simulink model "fft_biplex_test"  (Simulink 7.4)
settings: Solver=VariableStepDiscrete  StartTime=0.0  StopTime=2000  RelTol=1e-3
libraries: xbsIndex_r4 x808, casper_library_misc x46, casper_library_delays x10, casper_library_reorder x2, casper_library_ffts_twiddle x1
(part 2 of 8)

== system fft_biplex_test/fft_biplex/biplex_core/fft_stage_1 ==
  in1 : Inport  OutDataType=sfix(16)  OutScaling=2^0
  in2 : Inport  Port=2  OutDataType=sfix(16)  OutScaling=2^0
  of_in : Inport  Port=3  OutDataType=sfix(16)  OutScaling=2^0
  sync : Inport  Port=4  OutDataType=sfix(16)  OutScaling=2^0
  shift : Inport  Port=5  OutDataType=sfix(16)  OutScaling=2^0
  Counter : xbsIndex_r4/Counter  cnt_type=Free Running  cnt_to=Inf  operation=Up  start_count=0  cnt_by_val=1  arith_type=Unsigned  n_bits=FFTSize-FFTStage+1  bin_pt=0  load_pin=off  rst=on  en=off  explicit_period=off  period=1  dbl_ovrd=off  use_behavioral_HDL=off  implementation=Fabric  use_rpm=off  block_type=counter
      settings: xl_area=[0, 0, 0, 0, 0, 0, 0]  block_version=9.1.01
  Delay : xbsIndex_r4/Delay  en=off  latency=1  dbl_ovrd=off  reg_retiming=off  block_type=delay
      settings: xl_area=[0, 0, 0, 0, 0, 0, 0]  block_version=9.1.01
  Logical1 : xbsIndex_r4/Logical  logical_function=OR  inputs=2  en=off  latency=1  precision=Full  arith_type=Unsigned  n_bits=8  bin_pt=2  align_bp=on  dbl_ovrd=off  block_type=logical
      settings: xl_area=[0, 0, 0, 0, 0, 0, 0]  block_version=9.1.01
  Mux : xbsIndex_r4/Mux  inputs=2  en=off  latency=1  precision=Full  arith_type="Signed  (2's comp)"  n_bits=8  bin_pt=2  quantization=Truncate  overflow=Wrap  dbl_ovrd=off  block_type=mux
      settings: xl_area=[0, 0, 0, 0, 0, 0, 0]  block_version=9.1.01
  Mux1 : xbsIndex_r4/Mux  inputs=2  en=off  latency=1  precision=Full  arith_type="Signed  (2's comp)"  n_bits=8  bin_pt=2  quantization=Truncate  overflow=Wrap  dbl_ovrd=off  block_type=mux
      settings: xl_area=[0, 0, 0, 0, 0, 0, 0]  block_version=9.1.01
  Slice : xbsIndex_r4/Slice  nbits=1  boolean_output=on  mode=Lower Bit Location + Width  bit1=-(FFTStage - 1)  base1=MSB of Input  bit0=FFTStage - 1  base0=LSB of Input  dbl_ovrd=off  block_type=slice
      settings: infoedit="Extracts a given range of bits from each input sample and presents it at the output.  The output type is ordinarily unsigned with binary point at zero, but can be Boolean when the slice is one bit wide.<P><P>Hardware notes: In hardware this block costs nothing."  block_version=9.1.01
  Slice1 : xbsIndex_r4/Slice  nbits=1  boolean_output=off  mode=Upper Bit Location + Width  bit1=0  base1=MSB of Input  bit0=0  base0=LSB of Input  dbl_ovrd=off  block_type=slice
      settings: infoedit="Extracts a given range of bits from each input sample and presents it at the output.  The output type is ordinarily unsigned with binary point at zero, but can be Boolean when the slice is one bit wide.<P><P>Hardware notes: In hardware this block costs nothing."  block_version=9.1.01
  butterfly_direct : Subsystem  AncestorBlock=casper_library_ffts/butterfly_direct  mask(butterfly_direct){biplex=on, FFTSize=8, Coeffs=0, StepPeriod=7, coeff_bit_width=12, input_bit_width=12, downshift=off, add_latency=2, mult_latency=3, bram_latency=2, conv_latency=2, quantization=Round  (unbiased: +/- Inf), overflow=Saturate, arch=Virtex2Pro, opt_target=multipliers, coeffs_bram=off, use_hdl=on, use_embedded=off, hardcode_shifts=off, dsp48_adders=off}
      mask prompts: biplex "Used in biplex FFT"; FFTSize "Size of FFT: (2^? pts)"; Coeffs "Coefficients: (0 to 2^(FFTSize-1)-1)"; StepPeriod "Coefficient Step Period: (2^?)"; coeff_bit_width "Coefficient Bit Width"; input_bit_width "Input/Output Bit Width:"; add_latency "Add Latency"; mult_latency "Mult Latency"; bram_latency "BRAM Latency"; conv_latency "Convert latency"; quantization "Quantization Behavior"; overflow "Overflow Behavior"; arch "Architecture"; opt_target "Use less"; coeffs_bram "Store coefficients in BRAM"; use_hdl "Use behavioural HDL for multipliers"; use_embedded "Use embedded multipliers"; hardcode_shifts "Hardcode shift schedule"; dsp48_adders "Use DSP48s for adders"
      mask help: FFT internal block.
      mask init:
      | butterfly_direct_init(gcb, ...
      |     'biplex', biplex, ...
      |     'FFTSize', FFTSize, ...
      |     'Coeffs', Coeffs, ...
      |     'StepPeriod', StepPeriod, ...
      |     'coeff_bit_width', coeff_bit_width, ...
      |     'input_bit_width', input_bit_width, ...
      |     'hardcode_shifts', hardcode_shifts, ...
      |     'downshift', downshift, ...
      |     'add_latency', add_latency, ...
      |     'mult_latency', mult_latency, ...
      |     'bram_latency', bram_latency, ...
      |     'conv_latency', conv_latency, ...
      |     'quantization', quantization, ...
      |     'overflow', overflow, ...
      |     'arch', arch, ...
      |     'opt_target', opt_target, ...
      |     'coeffs_bram', coeffs_bram, ...    
      |     'use_hdl', use_hdl, ...
      |     'use_embedded', use_embedded, ...
      |     'dsp48_adders', dsp48_adders);
      settings: AttributesFormatString=|
      | twiddle_pass_through
      | coeffs in slices
      mask StyleString: checkbox,edit,edit,edit,edit,edit,checkbox,edit,edit,edit,edit,popup(Truncate|Round  (unbiased: +/- Inf)|Round  (unbiased: Even Values)),popup(Wrap|Saturate|Error),popup(Virtex2Pro|Virtex5),popup(logic|multipliers),checkbox,checkbox,checkbox,checkbox,checkbox
      mask CallbackString:
      | ||Coeffs = get_param(gcb, 'Coeffs');
      | if (length(eval(Coeffs)) == 1),
      |     set_param_state(gcb, 'StepPeriod', 'off');
      |     set_param_state(gcb, 'coeffs_bram', 'off');
      |     set_param_state(gcb, 'coeff_bit_width', 'off');
      | else
      |     set_param_state(gcb, 'StepPeriod', 'on');
      |     set_param_state(gcb, 'coeffs_bram', 'on');
      |     set_param_state(gcb, 'coeff_bit_width', 'on');
      | end|||||||||||fft_callback_arch(gcb);|||% make mutually exclusive with use_embedded.
      | 
      | use_hdl = get_param(gcb, 'use_hdl');
      | if strcmp(use_hdl, 'on'),
      |     set_param_state(gcb, 'use_embedded', 'off');
      | else
      |     set_param_state(gcb, 'use_embedded', 'on');
      | end|% make mutually exclusive with use_hdl.
      | 
      | use_hdl = get_param(gcb, 'use_embedded');
      | if strcmp(use_hdl, 'on'),
      |     set_param_state(gcb, 'use_hdl', 'off');
      | else
      |     set_param_state(gcb, 'use_hdl', 'on');
      | end|hardcode_shifts = get_param(gcb, 'hardcode_shifts');
      | set_param_state(gcb, 'downshift', hardcode_shifts);|fft_callback_dsp48_adders(gcb);
      mask TabNameString: Basic,Basic,Basic,Basic,Basic,Basic,Basic,Latency,Latency,Latency,Latency,Implementation,Implementation,Implementation,Implementation,Implementation,Implementation,Implementation,Implementation,Implementation
  delay_b : Subsystem  AncestorBlock=casper_library_delays/delay_bram  mask(delay_bram){DelayLen=2^(FFTSize-FFTStage), bram_latency=bram_latency, use_dsp48=off}
      mask prompts: DelayLen "Delay By:"; bram_latency "BRAM Latency"; use_dsp48 "Use DSP48"
      mask help: A delay block that uses BRAM for its storage.
      mask init:
      | if (DelayLen <= bram_latency)
      | 	error('delay value must be greater than BRAM Latency');
      | end
      | BitWidth = max(ceil(log2(DelayLen)), 2);
      | if strcmp(use_dsp48,'on'),
      |     set_param([gcb,'/Counter'], 'use_behavioral_HDL', 'off', ...
      |         'use_rpm', 'on', 'implementation', 'DSP48');
      | else, %default counter settings
      |         set_param([gcb,'/Counter'], 'use_behavioral_HDL', 'off', ...
      |         'use_rpm', 'off', 'implementation', 'Fabric');
      | end
      mask Help: eval('xlWeb(''http://casper.berkeley.edu/wiki/Delay_bram'')')
  delay_f : Subsystem  AncestorBlock=casper_library_delays/delay_bram  mask(delay_bram){DelayLen=2^(FFTSize-FFTStage), bram_latency=bram_latency, use_dsp48=off}
      mask prompts: DelayLen "Delay By:"; bram_latency "BRAM Latency"; use_dsp48 "Use DSP48"
      mask help: A delay block that uses BRAM for its storage.
      mask init: same as fft_biplex_test/fft_biplex/biplex_core/fft_stage_1/delay_b
      mask Help: eval('xlWeb(''http://casper.berkeley.edu/wiki/Delay_bram'')')
  sync_delay : casper_library_delays/sync_delay  SystemSampleTime=-1  DelayLen=2^(FFTSize - FFTStage)
  out1 : Outport  OutDataType=sfix(16)  OutScaling=2^0
  out2 : Outport  Port=2  OutDataType=sfix(16)  OutScaling=2^0
  of : Outport  Port=3  OutDataType=sfix(16)  OutScaling=2^0
  sync_out : Outport  Port=4  OutDataType=sfix(16)  OutScaling=2^0
  wires:
  butterfly_direct/4(sync_out) -> sync_out/1
  butterfly_direct/3(of) -> Logical1/1
  butterfly_direct/2(a-bw) -> out2/1
  butterfly_direct/1(a+bw) -> out1/1
  Slice/1 -> butterfly_direct/4(shift)
  sync_delay/1 -> butterfly_direct/3(sync)
  delay_b/1(Out1) -> butterfly_direct/1(a)
  in2/1 -> delay_f/1(In1)
  Slice1/1 -> Mux1/1, Mux/1
  in1/1 -> Mux1/2, Mux/3
  delay_f/1(Out1) -> Mux/2, Mux1/3
  Mux1/1 -> delay_b/1(In1)
  Mux/1 -> butterfly_direct/2(b)
  Counter/1 -> Slice1/1
  sync/1 -> Delay/1, Counter/1
  Delay/1 -> sync_delay/1
  Logical1/1 -> of/1
  of_in/1 -> Logical1/2
  shift/1 -> Slice/1

== system fft_biplex_test/fft_biplex/biplex_core/fft_stage_2 ==
  in1 : Inport  OutDataType=sfix(16)  OutScaling=2^0
  in2 : Inport  Port=2  OutDataType=sfix(16)  OutScaling=2^0
  of_in : Inport  Port=3  OutDataType=sfix(16)  OutScaling=2^0
  sync : Inport  Port=4  OutDataType=sfix(16)  OutScaling=2^0
  shift : Inport  Port=5  OutDataType=sfix(16)  OutScaling=2^0
  Counter : xbsIndex_r4/Counter  cnt_type=Free Running  cnt_to=Inf  operation=Up  start_count=0  cnt_by_val=1  arith_type=Unsigned  n_bits=FFTSize-FFTStage+1  bin_pt=0  load_pin=off  rst=on  en=off  explicit_period=off  period=1  dbl_ovrd=off  use_behavioral_HDL=off  implementation=Fabric  use_rpm=off  block_type=counter
      settings: xl_area=[0, 0, 0, 0, 0, 0, 0]  block_version=9.1.01
  Delay : xbsIndex_r4/Delay  en=off  latency=1  dbl_ovrd=off  reg_retiming=off  block_type=delay
      settings: xl_area=[0, 0, 0, 0, 0, 0, 0]  block_version=9.1.01
  Logical1 : xbsIndex_r4/Logical  logical_function=OR  inputs=2  en=off  latency=1  precision=Full  arith_type=Unsigned  n_bits=8  bin_pt=2  align_bp=on  dbl_ovrd=off  block_type=logical
      settings: xl_area=[0, 0, 0, 0, 0, 0, 0]  block_version=9.1.01
  Mux : xbsIndex_r4/Mux  inputs=2  en=off  latency=1  precision=Full  arith_type="Signed  (2's comp)"  n_bits=8  bin_pt=2  quantization=Truncate  overflow=Wrap  dbl_ovrd=off  block_type=mux
      settings: xl_area=[0, 0, 0, 0, 0, 0, 0]  block_version=9.1.01
  Mux1 : xbsIndex_r4/Mux  inputs=2  en=off  latency=1  precision=Full  arith_type="Signed  (2's comp)"  n_bits=8  bin_pt=2  quantization=Truncate  overflow=Wrap  dbl_ovrd=off  block_type=mux
      settings: xl_area=[0, 0, 0, 0, 0, 0, 0]  block_version=9.1.01
  Slice : xbsIndex_r4/Slice  nbits=1  boolean_output=on  mode=Lower Bit Location + Width  bit1=-(FFTStage - 1)  base1=MSB of Input  bit0=FFTStage - 1  base0=LSB of Input  dbl_ovrd=off  block_type=slice
      settings: infoedit="Extracts a given range of bits from each input sample and presents it at the output.  The output type is ordinarily unsigned with binary point at zero, but can be Boolean when the slice is one bit wide.<P><P>Hardware notes: In hardware this block costs nothing."  block_version=9.1.01
  Slice1 : xbsIndex_r4/Slice  nbits=1  boolean_output=off  mode=Upper Bit Location + Width  bit1=0  base1=MSB of Input  bit0=0  base0=LSB of Input  dbl_ovrd=off  block_type=slice
      settings: infoedit="Extracts a given range of bits from each input sample and presents it at the output.  The output type is ordinarily unsigned with binary point at zero, but can be Boolean when the slice is one bit wide.<P><P>Hardware notes: In hardware this block costs nothing."  block_version=9.1.01
  butterfly_direct : Subsystem  AncestorBlock=casper_library_ffts/butterfly_direct  mask(butterfly_direct){biplex=on, FFTSize=8, Coeffs=[0                                      1], StepPeriod=6, coeff_bit_width=12, input_bit_width=12, downshift=off, add_latency=2, mult_latency=3, bram_latency=2, conv_latency=2, quantization=Round  (unbiased: +/- Inf), overflow=Saturate, arch=Virtex2Pro, opt_target=multipliers, coeffs_bram=off, use_hdl=on, use_embedded=off, hardcode_shifts=off, dsp48_adders=off}
      mask prompts: biplex "Used in biplex FFT"; FFTSize "Size of FFT: (2^? pts)"; Coeffs "Coefficients: (0 to 2^(FFTSize-1)-1)"; StepPeriod "Coefficient Step Period: (2^?)"; coeff_bit_width "Coefficient Bit Width"; input_bit_width "Input/Output Bit Width:"; add_latency "Add Latency"; mult_latency "Mult Latency"; bram_latency "BRAM Latency"; conv_latency "Convert latency"; quantization "Quantization Behavior"; overflow "Overflow Behavior"; arch "Architecture"; opt_target "Use less"; coeffs_bram "Store coefficients in BRAM"; use_hdl "Use behavioural HDL for multipliers"; use_embedded "Use embedded multipliers"; hardcode_shifts "Hardcode shift schedule"; dsp48_adders "Use DSP48s for adders"
      mask help: FFT internal block.
      mask init: same as fft_biplex_test/fft_biplex/biplex_core/fft_stage_1/butterfly_direct
      settings: AttributesFormatString=|
      | twiddle_stage_2
      | coeffs in slices
      mask StyleString: checkbox,edit,edit,edit,edit,edit,checkbox,edit,edit,edit,edit,popup(Truncate|Round  (unbiased: +/- Inf)|Round  (unbiased: Even Values)),popup(Wrap|Saturate|Error),popup(Virtex2Pro|Virtex5),popup(logic|multipliers),checkbox,checkbox,checkbox,checkbox,checkbox
      mask CallbackString:
      | ||Coeffs = get_param(gcb, 'Coeffs');
      | if (length(eval(Coeffs)) == 1),
      |     set_param_state(gcb, 'StepPeriod', 'off');
      |     set_param_state(gcb, 'coeffs_bram', 'off');
      |     set_param_state(gcb, 'coeff_bit_width', 'off');
      | else
      |     set_param_state(gcb, 'StepPeriod', 'on');
      |     set_param_state(gcb, 'coeffs_bram', 'on');
      |     set_param_state(gcb, 'coeff_bit_width', 'on');
      | end|||||||||||fft_callback_arch(gcb);|||% make mutually exclusive with use_embedded.
      | 
      | use_hdl = get_param(gcb, 'use_hdl');
      | if strcmp(use_hdl, 'on'),
      |     set_param_state(gcb, 'use_embedded', 'off');
      | else
      |     set_param_state(gcb, 'use_embedded', 'on');
      | end|% make mutually exclusive with use_hdl.
      | 
      | use_hdl = get_param(gcb, 'use_embedded');
      | if strcmp(use_hdl, 'on'),
      |     set_param_state(gcb, 'use_hdl', 'off');
      | else
      |     set_param_state(gcb, 'use_hdl', 'on');
      | end|hardcode_shifts = get_param(gcb, 'hardcode_shifts');
      | set_param_state(gcb, 'downshift', hardcode_shifts);|fft_callback_dsp48_adders(gcb);
      mask TabNameString: Basic,Basic,Basic,Basic,Basic,Basic,Basic,Latency,Latency,Latency,Latency,Implementation,Implementation,Implementation,Implementation,Implementation,Implementation,Implementation,Implementation,Implementation
  delay_b : Subsystem  AncestorBlock=casper_library_delays/delay_bram  mask(delay_bram){DelayLen=2^(FFTSize-FFTStage), bram_latency=bram_latency, use_dsp48=off}
      mask prompts: DelayLen "Delay By:"; bram_latency "BRAM Latency"; use_dsp48 "Use DSP48"
      mask help: A delay block that uses BRAM for its storage.
      mask init: same as fft_biplex_test/fft_biplex/biplex_core/fft_stage_1/delay_b
      mask Help: eval('xlWeb(''http://casper.berkeley.edu/wiki/Delay_bram'')')
  delay_f : Subsystem  AncestorBlock=casper_library_delays/delay_bram  mask(delay_bram){DelayLen=2^(FFTSize-FFTStage), bram_latency=bram_latency, use_dsp48=off}
      mask prompts: DelayLen "Delay By:"; bram_latency "BRAM Latency"; use_dsp48 "Use DSP48"
      mask help: A delay block that uses BRAM for its storage.
      mask init: same as fft_biplex_test/fft_biplex/biplex_core/fft_stage_1/delay_b
      mask Help: eval('xlWeb(''http://casper.berkeley.edu/wiki/Delay_bram'')')
  sync_delay : casper_library_delays/sync_delay  SystemSampleTime=-1  DelayLen=2^(FFTSize - FFTStage)
  out1 : Outport  OutDataType=sfix(16)  OutScaling=2^0
  out2 : Outport  Port=2  OutDataType=sfix(16)  OutScaling=2^0
  of : Outport  Port=3  OutDataType=sfix(16)  OutScaling=2^0
  sync_out : Outport  Port=4  OutDataType=sfix(16)  OutScaling=2^0
  wires:
  butterfly_direct/4(sync_out) -> sync_out/1
  butterfly_direct/3(of) -> Logical1/1
  butterfly_direct/2(a-bw) -> out2/1
  butterfly_direct/1(a+bw) -> out1/1
  Slice/1 -> butterfly_direct/4(shift)
  sync_delay/1 -> butterfly_direct/3(sync)
  delay_b/1(Out1) -> butterfly_direct/1(a)
  in2/1 -> delay_f/1(In1)
  Slice1/1 -> Mux1/1, Mux/1
  in1/1 -> Mux1/2, Mux/3
  delay_f/1(Out1) -> Mux/2, Mux1/3
  Mux1/1 -> delay_b/1(In1)
  Mux/1 -> butterfly_direct/2(b)
  Counter/1 -> Slice1/1
  sync/1 -> Delay/1, Counter/1
  Delay/1 -> sync_delay/1
  Logical1/1 -> of/1
  of_in/1 -> Logical1/2
  shift/1 -> Slice/1

== system fft_biplex_test/fft_biplex/biplex_core/fft_stage_3 ==
  in1 : Inport  OutDataType=sfix(16)  OutScaling=2^0
  in2 : Inport  Port=2  OutDataType=sfix(16)  OutScaling=2^0
  of_in : Inport  Port=3  OutDataType=sfix(16)  OutScaling=2^0
  sync : Inport  Port=4  OutDataType=sfix(16)  OutScaling=2^0
  shift : Inport  Port=5  OutDataType=sfix(16)  OutScaling=2^0
  Counter : xbsIndex_r4/Counter  cnt_type=Free Running  cnt_to=Inf  operation=Up  start_count=0  cnt_by_val=1  arith_type=Unsigned  n_bits=FFTSize-FFTStage+1  bin_pt=0  load_pin=off  rst=on  en=off  explicit_period=off  period=1  dbl_ovrd=off  use_behavioral_HDL=off  implementation=Fabric  use_rpm=off  block_type=counter
      settings: xl_area=[0, 0, 0, 0, 0, 0, 0]  block_version=9.1.01
  Delay : xbsIndex_r4/Delay  en=off  latency=1  dbl_ovrd=off  reg_retiming=off  block_type=delay
      settings: xl_area=[0, 0, 0, 0, 0, 0, 0]  block_version=9.1.01
  Logical1 : xbsIndex_r4/Logical  logical_function=OR  inputs=2  en=off  latency=1  precision=Full  arith_type=Unsigned  n_bits=8  bin_pt=2  align_bp=on  dbl_ovrd=off  block_type=logical
      settings: xl_area=[0, 0, 0, 0, 0, 0, 0]  block_version=9.1.01
  Mux : xbsIndex_r4/Mux  inputs=2  en=off  latency=1  precision=Full  arith_type="Signed  (2's comp)"  n_bits=8  bin_pt=2  quantization=Truncate  overflow=Wrap  dbl_ovrd=off  block_type=mux
      settings: xl_area=[0, 0, 0, 0, 0, 0, 0]  block_version=9.1.01
  Mux1 : xbsIndex_r4/Mux  inputs=2  en=off  latency=1  precision=Full  arith_type="Signed  (2's comp)"  n_bits=8  bin_pt=2  quantization=Truncate  overflow=Wrap  dbl_ovrd=off  block_type=mux
      settings: xl_area=[0, 0, 0, 0, 0, 0, 0]  block_version=9.1.01
  Slice : xbsIndex_r4/Slice  nbits=1  boolean_output=on  mode=Lower Bit Location + Width  bit1=-(FFTStage - 1)  base1=MSB of Input  bit0=FFTStage - 1  base0=LSB of Input  dbl_ovrd=off  block_type=slice
      settings: infoedit="Extracts a given range of bits from each input sample and presents it at the output.  The output type is ordinarily unsigned with binary point at zero, but can be Boolean when the slice is one bit wide.<P><P>Hardware notes: In hardware this block costs nothing."  block_version=9.1.01
  Slice1 : xbsIndex_r4/Slice  nbits=1  boolean_output=off  mode=Upper Bit Location + Width  bit1=0  base1=MSB of Input  bit0=0  base0=LSB of Input  dbl_ovrd=off  block_type=slice
      settings: infoedit="Extracts a given range of bits from each input sample and presents it at the output.  The output type is ordinarily unsigned with binary point at zero, but can be Boolean when the slice is one bit wide.<P><P>Hardware notes: In hardware this block costs nothing."  block_version=9.1.01
  butterfly_direct : Subsystem  AncestorBlock=casper_library_ffts/butterfly_direct  mask(butterfly_direct){biplex=on, FFTSize=8, Coeffs=getfield( getfield( get_param( gcb,'UserData' ), 'parameters'),'Coeffs'), StepPeriod=5, coeff_bit_width=12, input_bit_width=12, downshift=off, add_latency=2, mult_latency=3, bram_latency=2, conv_latency=2, quantization=Round  (unbiased: +/- Inf), overflow=Saturate, arch=Virtex2Pro, opt_target=multipliers, coeffs_bram=on, use_hdl=on, use_embedded=off, hardcode_shifts=off, dsp48_adders=off}
      mask prompts: biplex "Used in biplex FFT"; FFTSize "Size of FFT: (2^? pts)"; Coeffs "Coefficients: (0 to 2^(FFTSize-1)-1)"; StepPeriod "Coefficient Step Period: (2^?)"; coeff_bit_width "Coefficient Bit Width"; input_bit_width "Input/Output Bit Width:"; add_latency "Add Latency"; mult_latency "Mult Latency"; bram_latency "BRAM Latency"; conv_latency "Convert latency"; quantization "Quantization Behavior"; overflow "Overflow Behavior"; arch "Architecture"; opt_target "Use less"; coeffs_bram "Store coefficients in BRAM"; use_hdl "Use behavioural HDL for multipliers"; use_embedded "Use embedded multipliers"; hardcode_shifts "Hardcode shift schedule"; dsp48_adders "Use DSP48s for adders"
      mask help: FFT internal block.
      mask init: same as fft_biplex_test/fft_biplex/biplex_core/fft_stage_1/butterfly_direct
      settings: AttributesFormatString=|
      | twiddle_general_3mult
      | coeffs in BRAM
      mask StyleString: checkbox,edit,edit,edit,edit,edit,checkbox,edit,edit,edit,edit,popup(Truncate|Round  (unbiased: +/- Inf)|Round  (unbiased: Even Values)),popup(Wrap|Saturate|Error),popup(Virtex2Pro|Virtex5),popup(logic|multipliers),checkbox,checkbox,checkbox,checkbox,checkbox
      mask CallbackString:
      | ||Coeffs = get_param(gcb, 'Coeffs');
      | if (length(eval(Coeffs)) == 1),
      |     set_param_state(gcb, 'StepPeriod', 'off');
      |     set_param_state(gcb, 'coeffs_bram', 'off');
      |     set_param_state(gcb, 'coeff_bit_width', 'off');
      | else
      |     set_param_state(gcb, 'StepPeriod', 'on');
      |     set_param_state(gcb, 'coeffs_bram', 'on');
      |     set_param_state(gcb, 'coeff_bit_width', 'on');
      | end|||||||||||fft_callback_arch(gcb);|||% make mutually exclusive with use_embedded.
      | 
      | use_hdl = get_param(gcb, 'use_hdl');
      | if strcmp(use_hdl, 'on'),
      |     set_param_state(gcb, 'use_embedded', 'off');
      | else
      |     set_param_state(gcb, 'use_embedded', 'on');
      | end|% make mutually exclusive with use_hdl.
      | 
      | use_hdl = get_param(gcb, 'use_embedded');
      | if strcmp(use_hdl, 'on'),
      |     set_param_state(gcb, 'use_hdl', 'off');
      | else
      |     set_param_state(gcb, 'use_hdl', 'on');
      | end|hardcode_shifts = get_param(gcb, 'hardcode_shifts');
      | set_param_state(gcb, 'downshift', hardcode_shifts);|fft_callback_dsp48_adders(gcb);
      mask TabNameString: Basic,Basic,Basic,Basic,Basic,Basic,Basic,Latency,Latency,Latency,Latency,Implementation,Implementation,Implementation,Implementation,Implementation,Implementation,Implementation,Implementation,Implementation
  delay_b : Subsystem  AncestorBlock=casper_library_delays/delay_bram  mask(delay_bram){DelayLen=2^(FFTSize-FFTStage), bram_latency=bram_latency, use_dsp48=off}
      mask prompts: DelayLen "Delay By:"; bram_latency "BRAM Latency"; use_dsp48 "Use DSP48"
      mask help: A delay block that uses BRAM for its storage.
      mask init: same as fft_biplex_test/fft_biplex/biplex_core/fft_stage_1/delay_b
      mask Help: eval('xlWeb(''http://casper.berkeley.edu/wiki/Delay_bram'')')
  delay_f : Subsystem  AncestorBlock=casper_library_delays/delay_bram  mask(delay_bram){DelayLen=2^(FFTSize-FFTStage), bram_latency=bram_latency, use_dsp48=off}
      mask prompts: DelayLen "Delay By:"; bram_latency "BRAM Latency"; use_dsp48 "Use DSP48"
      mask help: A delay block that uses BRAM for its storage.
      mask init: same as fft_biplex_test/fft_biplex/biplex_core/fft_stage_1/delay_b
      mask Help: eval('xlWeb(''http://casper.berkeley.edu/wiki/Delay_bram'')')
  sync_delay : casper_library_delays/sync_delay  SystemSampleTime=-1  DelayLen=2^(FFTSize - FFTStage)
  out1 : Outport  OutDataType=sfix(16)  OutScaling=2^0
  out2 : Outport  Port=2  OutDataType=sfix(16)  OutScaling=2^0
  of : Outport  Port=3  OutDataType=sfix(16)  OutScaling=2^0
  sync_out : Outport  Port=4  OutDataType=sfix(16)  OutScaling=2^0
  wires:
  shift/1 -> Slice/1
  of_in/1 -> Logical1/2
  Logical1/1 -> of/1
  Delay/1 -> sync_delay/1
  sync/1 -> Counter/1, Delay/1
  Counter/1 -> Slice1/1
  Mux/1 -> butterfly_direct/2(b)
  Mux1/1 -> delay_b/1(In1)
  delay_f/1(Out1) -> Mux1/3, Mux/2
  in1/1 -> Mux/3, Mux1/2
  Slice1/1 -> Mux/1, Mux1/1
  in2/1 -> delay_f/1(In1)
  delay_b/1(Out1) -> butterfly_direct/1(a)
  sync_delay/1 -> butterfly_direct/3(sync)
  Slice/1 -> butterfly_direct/4(shift)
  butterfly_direct/1(a+bw) -> out1/1
  butterfly_direct/2(a-bw) -> out2/1
  butterfly_direct/3(of) -> Logical1/1
  butterfly_direct/4(sync_out) -> sync_out/1

== system fft_biplex_test/fft_biplex/biplex_core/fft_stage_4 ==
  in1 : Inport  OutDataType=sfix(16)  OutScaling=2^0
  in2 : Inport  Port=2  OutDataType=sfix(16)  OutScaling=2^0
  of_in : Inport  Port=3  OutDataType=sfix(16)  OutScaling=2^0
  sync : Inport  Port=4  OutDataType=sfix(16)  OutScaling=2^0
  shift : Inport  Port=5  OutDataType=sfix(16)  OutScaling=2^0
  Counter : xbsIndex_r4/Counter  cnt_type=Free Running  cnt_to=Inf  operation=Up  start_count=0  cnt_by_val=1  arith_type=Unsigned  n_bits=FFTSize-FFTStage+1  bin_pt=0  load_pin=off  rst=on  en=off  explicit_period=off  period=1  dbl_ovrd=off  use_behavioral_HDL=off  implementation=Fabric  use_rpm=off  block_type=counter
      settings: xl_area=[0, 0, 0, 0, 0, 0, 0]  block_version=9.1.01
  Delay : xbsIndex_r4/Delay  en=off  latency=1  dbl_ovrd=off  reg_retiming=off  block_type=delay
      settings: xl_area=[0, 0, 0, 0, 0, 0, 0]  block_version=9.1.01
  Logical1 : xbsIndex_r4/Logical  logical_function=OR  inputs=2  en=off  latency=1  precision=Full  arith_type=Unsigned  n_bits=8  bin_pt=2  align_bp=on  dbl_ovrd=off  block_type=logical
      settings: xl_area=[0, 0, 0, 0, 0, 0, 0]  block_version=9.1.01
  Mux : xbsIndex_r4/Mux  inputs=2  en=off  latency=1  precision=Full  arith_type="Signed  (2's comp)"  n_bits=8  bin_pt=2  quantization=Truncate  overflow=Wrap  dbl_ovrd=off  block_type=mux
      settings: xl_area=[0, 0, 0, 0, 0, 0, 0]  block_version=9.1.01
  Mux1 : xbsIndex_r4/Mux  inputs=2  en=off  latency=1  precision=Full  arith_type="Signed  (2's comp)"  n_bits=8  bin_pt=2  quantization=Truncate  overflow=Wrap  dbl_ovrd=off  block_type=mux
      settings: xl_area=[0, 0, 0, 0, 0, 0, 0]  block_version=9.1.01
  Slice : xbsIndex_r4/Slice  nbits=1  boolean_output=on  mode=Lower Bit Location + Width  bit1=-(FFTStage - 1)  base1=MSB of Input  bit0=FFTStage - 1  base0=LSB of Input  dbl_ovrd=off  block_type=slice
      settings: infoedit="Extracts a given range of bits from each input sample and presents it at the output.  The output type is ordinarily unsigned with binary point at zero, but can be Boolean when the slice is one bit wide.<P><P>Hardware notes: In hardware this block costs nothing."  block_version=9.1.01
  Slice1 : xbsIndex_r4/Slice  nbits=1  boolean_output=off  mode=Upper Bit Location + Width  bit1=0  base1=MSB of Input  bit0=0  base0=LSB of Input  dbl_ovrd=off  block_type=slice
      settings: infoedit="Extracts a given range of bits from each input sample and presents it at the output.  The output type is ordinarily unsigned with binary point at zero, but can be Boolean when the slice is one bit wide.<P><P>Hardware notes: In hardware this block costs nothing."  block_version=9.1.01
  butterfly_direct : Subsystem  AncestorBlock=casper_library_ffts/butterfly_direct  mask(butterfly_direct){biplex=on, FFTSize=8, Coeffs=getfield( getfield( get_param( gcb,'UserData' ), 'parameters'),'Coeffs'), StepPeriod=4, coeff_bit_width=12, input_bit_width=12, downshift=off, add_latency=2, mult_latency=3, bram_latency=2, conv_latency=2, quantization=Round  (unbiased: +/- Inf), overflow=Saturate, arch=Virtex2Pro, opt_target=multipliers, coeffs_bram=on, use_hdl=on, use_embedded=off, hardcode_shifts=off, dsp48_adders=off}
      mask prompts: biplex "Used in biplex FFT"; FFTSize "Size of FFT: (2^? pts)"; Coeffs "Coefficients: (0 to 2^(FFTSize-1)-1)"; StepPeriod "Coefficient Step Period: (2^?)"; coeff_bit_width "Coefficient Bit Width"; input_bit_width "Input/Output Bit Width:"; add_latency "Add Latency"; mult_latency "Mult Latency"; bram_latency "BRAM Latency"; conv_latency "Convert latency"; quantization "Quantization Behavior"; overflow "Overflow Behavior"; arch "Architecture"; opt_target "Use less"; coeffs_bram "Store coefficients in BRAM"; use_hdl "Use behavioural HDL for multipliers"; use_embedded "Use embedded multipliers"; hardcode_shifts "Hardcode shift schedule"; dsp48_adders "Use DSP48s for adders"
      mask help: FFT internal block.
      mask init: same as fft_biplex_test/fft_biplex/biplex_core/fft_stage_1/butterfly_direct
      settings: AttributesFormatString=|
      | twiddle_general_3mult
      | coeffs in BRAM
      mask StyleString: checkbox,edit,edit,edit,edit,edit,checkbox,edit,edit,edit,edit,popup(Truncate|Round  (unbiased: +/- Inf)|Round  (unbiased: Even Values)),popup(Wrap|Saturate|Error),popup(Virtex2Pro|Virtex5),popup(logic|multipliers),checkbox,checkbox,checkbox,checkbox,checkbox
      mask CallbackString:
      | ||Coeffs = get_param(gcb, 'Coeffs');
      | if (length(eval(Coeffs)) == 1),
      |     set_param_state(gcb, 'StepPeriod', 'off');
      |     set_param_state(gcb, 'coeffs_bram', 'off');
      |     set_param_state(gcb, 'coeff_bit_width', 'off');
      | else
      |     set_param_state(gcb, 'StepPeriod', 'on');
      |     set_param_state(gcb, 'coeffs_bram', 'on');
      |     set_param_state(gcb, 'coeff_bit_width', 'on');
      | end|||||||||||fft_callback_arch(gcb);|||% make mutually exclusive with use_embedded.
      | 
      | use_hdl = get_param(gcb, 'use_hdl');
      | if strcmp(use_hdl, 'on'),
      |     set_param_state(gcb, 'use_embedded', 'off');
      | else
      |     set_param_state(gcb, 'use_embedded', 'on');
      | end|% make mutually exclusive with use_hdl.
      | 
      | use_hdl = get_param(gcb, 'use_embedded');
      | if strcmp(use_hdl, 'on'),
      |     set_param_state(gcb, 'use_hdl', 'off');
      | else
      |     set_param_state(gcb, 'use_hdl', 'on');
      | end|hardcode_shifts = get_param(gcb, 'hardcode_shifts');
      | set_param_state(gcb, 'downshift', hardcode_shifts);|fft_callback_dsp48_adders(gcb);
      mask TabNameString: Basic,Basic,Basic,Basic,Basic,Basic,Basic,Latency,Latency,Latency,Latency,Implementation,Implementation,Implementation,Implementation,Implementation,Implementation,Implementation,Implementation,Implementation
  delay_b : Subsystem  AncestorBlock=casper_library_delays/delay_bram  mask(delay_bram){DelayLen=2^(FFTSize-FFTStage), bram_latency=bram_latency, use_dsp48=off}
      mask prompts: DelayLen "Delay By:"; bram_latency "BRAM Latency"; use_dsp48 "Use DSP48"
      mask help: A delay block that uses BRAM for its storage.
      mask init: same as fft_biplex_test/fft_biplex/biplex_core/fft_stage_1/delay_b
      mask Help: eval('xlWeb(''http://casper.berkeley.edu/wiki/Delay_bram'')')
  delay_f : Subsystem  AncestorBlock=casper_library_delays/delay_bram  mask(delay_bram){DelayLen=2^(FFTSize-FFTStage), bram_latency=bram_latency, use_dsp48=off}
      mask prompts: DelayLen "Delay By:"; bram_latency "BRAM Latency"; use_dsp48 "Use DSP48"
      mask help: A delay block that uses BRAM for its storage.
      mask init: same as fft_biplex_test/fft_biplex/biplex_core/fft_stage_1/delay_b
      mask Help: eval('xlWeb(''http://casper.berkeley.edu/wiki/Delay_bram'')')
  sync_delay : casper_library_delays/sync_delay  SystemSampleTime=-1  DelayLen=2^(FFTSize - FFTStage)
  out1 : Outport  OutDataType=sfix(16)  OutScaling=2^0
  out2 : Outport  Port=2  OutDataType=sfix(16)  OutScaling=2^0
  of : Outport  Port=3  OutDataType=sfix(16)  OutScaling=2^0
  sync_out : Outport  Port=4  OutDataType=sfix(16)  OutScaling=2^0
  wires:
  shift/1 -> Slice/1
  of_in/1 -> Logical1/2
  Logical1/1 -> of/1
  Delay/1 -> sync_delay/1
  sync/1 -> Counter/1, Delay/1
  Counter/1 -> Slice1/1
  Mux/1 -> butterfly_direct/2(b)
  Mux1/1 -> delay_b/1(In1)
  delay_f/1(Out1) -> Mux1/3, Mux/2
  in1/1 -> Mux/3, Mux1/2
  Slice1/1 -> Mux/1, Mux1/1
  in2/1 -> delay_f/1(In1)
  delay_b/1(Out1) -> butterfly_direct/1(a)
  sync_delay/1 -> butterfly_direct/3(sync)
  Slice/1 -> butterfly_direct/4(shift)
  butterfly_direct/1(a+bw) -> out1/1
  butterfly_direct/2(a-bw) -> out2/1
  butterfly_direct/3(of) -> Logical1/1
  butterfly_direct/4(sync_out) -> sync_out/1

== system fft_biplex_test/fft_biplex/biplex_core/fft_stage_5 ==
  in1 : Inport  OutDataType=sfix(16)  OutScaling=2^0
  in2 : Inport  Port=2  OutDataType=sfix(16)  OutScaling=2^0
  of_in : Inport  Port=3  OutDataType=sfix(16)  OutScaling=2^0
  sync : Inport  Port=4  OutDataType=sfix(16)  OutScaling=2^0
  shift : Inport  Port=5  OutDataType=sfix(16)  OutScaling=2^0
  Counter : xbsIndex_r4/Counter  cnt_type=Free Running  cnt_to=Inf  operation=Up  start_count=0  cnt_by_val=1  arith_type=Unsigned  n_bits=FFTSize-FFTStage+1  bin_pt=0  load_pin=off  rst=on  en=off  explicit_period=off  period=1  dbl_ovrd=off  use_behavioral_HDL=off  implementation=Fabric  use_rpm=off  block_type=counter
      settings: xl_area=[0, 0, 0, 0, 0, 0, 0]  block_version=9.1.01
  Delay : xbsIndex_r4/Delay  en=off  latency=1  dbl_ovrd=off  reg_retiming=off  block_type=delay
      settings: xl_area=[0, 0, 0, 0, 0, 0, 0]  block_version=9.1.01
  Logical1 : xbsIndex_r4/Logical  logical_function=OR  inputs=2  en=off  latency=1  precision=Full  arith_type=Unsigned  n_bits=8  bin_pt=2  align_bp=on  dbl_ovrd=off  block_type=logical
      settings: xl_area=[0, 0, 0, 0, 0, 0, 0]  block_version=9.1.01
  Mux : xbsIndex_r4/Mux  inputs=2  en=off  latency=1  precision=Full  arith_type="Signed  (2's comp)"  n_bits=8  bin_pt=2  quantization=Truncate  overflow=Wrap  dbl_ovrd=off  block_type=mux
      settings: xl_area=[0, 0, 0, 0, 0, 0, 0]  block_version=9.1.01
  Mux1 : xbsIndex_r4/Mux  inputs=2  en=off  latency=1  precision=Full  arith_type="Signed  (2's comp)"  n_bits=8  bin_pt=2  quantization=Truncate  overflow=Wrap  dbl_ovrd=off  block_type=mux
      settings: xl_area=[0, 0, 0, 0, 0, 0, 0]  block_version=9.1.01
  Slice : xbsIndex_r4/Slice  nbits=1  boolean_output=on  mode=Lower Bit Location + Width  bit1=-(FFTStage - 1)  base1=MSB of Input  bit0=FFTStage - 1  base0=LSB of Input  dbl_ovrd=off  block_type=slice
      settings: infoedit="Extracts a given range of bits from each input sample and presents it at the output.  The output type is ordinarily unsigned with binary point at zero, but can be Boolean when the slice is one bit wide.<P><P>Hardware notes: In hardware this block costs nothing."  block_version=9.1.01
  Slice1 : xbsIndex_r4/Slice  nbits=1  boolean_output=off  mode=Upper Bit Location + Width  bit1=0  base1=MSB of Input  bit0=0  base0=LSB of Input  dbl_ovrd=off  block_type=slice
      settings: infoedit="Extracts a given range of bits from each input sample and presents it at the output.  The output type is ordinarily unsigned with binary point at zero, but can be Boolean when the slice is one bit wide.<P><P>Hardware notes: In hardware this block costs nothing."  block_version=9.1.01
  butterfly_direct : Subsystem  AncestorBlock=casper_library_ffts/butterfly_direct  mask(butterfly_direct){biplex=on, FFTSize=8, Coeffs=getfield( getfield( get_param( gcb,'UserData' ), 'parameters'),'Coeffs'), StepPeriod=3, coeff_bit_width=12, input_bit_width=12, downshift=off, add_latency=2, mult_latency=3, bram_latency=2, conv_latency=2, quantization=Round  (unbiased: +/- Inf), overflow=Saturate, arch=Virtex2Pro, opt_target=multipliers, coeffs_bram=on, use_hdl=on, use_embedded=off, hardcode_shifts=off, dsp48_adders=off}
      mask prompts: biplex "Used in biplex FFT"; FFTSize "Size of FFT: (2^? pts)"; Coeffs "Coefficients: (0 to 2^(FFTSize-1)-1)"; StepPeriod "Coefficient Step Period: (2^?)"; coeff_bit_width "Coefficient Bit Width"; input_bit_width "Input/Output Bit Width:"; add_latency "Add Latency"; mult_latency "Mult Latency"; bram_latency "BRAM Latency"; conv_latency "Convert latency"; quantization "Quantization Behavior"; overflow "Overflow Behavior"; arch "Architecture"; opt_target "Use less"; coeffs_bram "Store coefficients in BRAM"; use_hdl "Use behavioural HDL for multipliers"; use_embedded "Use embedded multipliers"; hardcode_shifts "Hardcode shift schedule"; dsp48_adders "Use DSP48s for adders"
      mask help: FFT internal block.
      mask init: same as fft_biplex_test/fft_biplex/biplex_core/fft_stage_1/butterfly_direct
      settings: AttributesFormatString=|
      | twiddle_general_3mult
      | coeffs in BRAM
      mask StyleString: checkbox,edit,edit,edit,edit,edit,checkbox,edit,edit,edit,edit,popup(Truncate|Round  (unbiased: +/- Inf)|Round  (unbiased: Even Values)),popup(Wrap|Saturate|Error),popup(Virtex2Pro|Virtex5),popup(logic|multipliers),checkbox,checkbox,checkbox,checkbox,checkbox
      mask CallbackString:
      | ||Coeffs = get_param(gcb, 'Coeffs');
      | if (length(eval(Coeffs)) == 1),
      |     set_param_state(gcb, 'StepPeriod', 'off');
      |     set_param_state(gcb, 'coeffs_bram', 'off');
      |     set_param_state(gcb, 'coeff_bit_width', 'off');
      | else
      |     set_param_state(gcb, 'StepPeriod', 'on');
      |     set_param_state(gcb, 'coeffs_bram', 'on');
      |     set_param_state(gcb, 'coeff_bit_width', 'on');
      | end|||||||||||fft_callback_arch(gcb);|||% make mutually exclusive with use_embedded.
      | 
      | use_hdl = get_param(gcb, 'use_hdl');
      | if strcmp(use_hdl, 'on'),
      |     set_param_state(gcb, 'use_embedded', 'off');
      | else
      |     set_param_state(gcb, 'use_embedded', 'on');
      | end|% make mutually exclusive with use_hdl.
      | 
      | use_hdl = get_param(gcb, 'use_embedded');
      | if strcmp(use_hdl, 'on'),
      |     set_param_state(gcb, 'use_hdl', 'off');
      | else
      |     set_param_state(gcb, 'use_hdl', 'on');
      | end|hardcode_shifts = get_param(gcb, 'hardcode_shifts');
      | set_param_state(gcb, 'downshift', hardcode_shifts);|fft_callback_dsp48_adders(gcb);
      mask TabNameString: Basic,Basic,Basic,Basic,Basic,Basic,Basic,Latency,Latency,Latency,Latency,Implementation,Implementation,Implementation,Implementation,Implementation,Implementation,Implementation,Implementation,Implementation
  delay_b : Subsystem  AncestorBlock=casper_library_delays/delay_bram  mask(delay_bram){DelayLen=2^(FFTSize-FFTStage), bram_latency=bram_latency, use_dsp48=off}
      mask prompts: DelayLen "Delay By:"; bram_latency "BRAM Latency"; use_dsp48 "Use DSP48"
      mask help: A delay block that uses BRAM for its storage.
      mask init: same as fft_biplex_test/fft_biplex/biplex_core/fft_stage_1/delay_b
      mask Help: eval('xlWeb(''http://casper.berkeley.edu/wiki/Delay_bram'')')
  delay_f : Subsystem  AncestorBlock=casper_library_delays/delay_bram  mask(delay_bram){DelayLen=2^(FFTSize-FFTStage), bram_latency=bram_latency, use_dsp48=off}
      mask prompts: DelayLen "Delay By:"; bram_latency "BRAM Latency"; use_dsp48 "Use DSP48"
      mask help: A delay block that uses BRAM for its storage.
      mask init: same as fft_biplex_test/fft_biplex/biplex_core/fft_stage_1/delay_b
      mask Help: eval('xlWeb(''http://casper.berkeley.edu/wiki/Delay_bram'')')
  sync_delay : casper_library_delays/sync_delay  SystemSampleTime=-1  DelayLen=2^(FFTSize - FFTStage)
  out1 : Outport  OutDataType=sfix(16)  OutScaling=2^0
  out2 : Outport  Port=2  OutDataType=sfix(16)  OutScaling=2^0
  of : Outport  Port=3  OutDataType=sfix(16)  OutScaling=2^0
  sync_out : Outport  Port=4  OutDataType=sfix(16)  OutScaling=2^0
  wires:
  shift/1 -> Slice/1
  of_in/1 -> Logical1/2
  Logical1/1 -> of/1
  Delay/1 -> sync_delay/1
  sync/1 -> Counter/1, Delay/1
  Counter/1 -> Slice1/1
  Mux/1 -> butterfly_direct/2(b)
  Mux1/1 -> delay_b/1(In1)
  delay_f/1(Out1) -> Mux1/3, Mux/2
  in1/1 -> Mux/3, Mux1/2
  Slice1/1 -> Mux/1, Mux1/1
  in2/1 -> delay_f/1(In1)
  delay_b/1(Out1) -> butterfly_direct/1(a)
  sync_delay/1 -> butterfly_direct/3(sync)
  Slice/1 -> butterfly_direct/4(shift)
  butterfly_direct/1(a+bw) -> out1/1
  butterfly_direct/2(a-bw) -> out2/1
  butterfly_direct/3(of) -> Logical1/1
  butterfly_direct/4(sync_out) -> sync_out/1

== system fft_biplex_test/fft_biplex/biplex_core/fft_stage_6 ==
  in1 : Inport  OutDataType=sfix(16)  OutScaling=2^0
  in2 : Inport  Port=2  OutDataType=sfix(16)  OutScaling=2^0
  of_in : Inport  Port=3  OutDataType=sfix(16)  OutScaling=2^0
  sync : Inport  Port=4  OutDataType=sfix(16)  OutScaling=2^0
  shift : Inport  Port=5  OutDataType=sfix(16)  OutScaling=2^0
  Counter : xbsIndex_r4/Counter  cnt_type=Free Running  cnt_to=Inf  operation=Up  start_count=0  cnt_by_val=1  arith_type=Unsigned  n_bits=FFTSize-FFTStage+1  bin_pt=0  load_pin=off  rst=on  en=off  explicit_period=off  period=1  dbl_ovrd=off  use_behavioral_HDL=off  implementation=Fabric  use_rpm=off  block_type=counter
      settings: xl_area=[0, 0, 0, 0, 0, 0, 0]  block_version=9.1.01
  Delay : xbsIndex_r4/Delay  en=off  latency=1  dbl_ovrd=off  reg_retiming=off  block_type=delay
      settings: xl_area=[0, 0, 0, 0, 0, 0, 0]  block_version=9.1.01
  Logical1 : xbsIndex_r4/Logical  logical_function=OR  inputs=2  en=off  latency=1  precision=Full  arith_type=Unsigned  n_bits=8  bin_pt=2  align_bp=on  dbl_ovrd=off  block_type=logical
      settings: xl_area=[0, 0, 0, 0, 0, 0, 0]  block_version=9.1.01
  Mux : xbsIndex_r4/Mux  inputs=2  en=off  latency=1  precision=Full  arith_type="Signed  (2's comp)"  n_bits=8  bin_pt=2  quantization=Truncate  overflow=Wrap  dbl_ovrd=off  block_type=mux
      settings: xl_area=[0, 0, 0, 0, 0, 0, 0]  block_version=9.1.01
  Mux1 : xbsIndex_r4/Mux  inputs=2  en=off  latency=1  precision=Full  arith_type="Signed  (2's comp)"  n_bits=8  bin_pt=2  quantization=Truncate  overflow=Wrap  dbl_ovrd=off  block_type=mux
      settings: xl_area=[0, 0, 0, 0, 0, 0, 0]  block_version=9.1.01
  Slice : xbsIndex_r4/Slice  nbits=1  boolean_output=on  mode=Lower Bit Location + Width  bit1=-(FFTStage - 1)  base1=MSB of Input  bit0=FFTStage - 1  base0=LSB of Input  dbl_ovrd=off  block_type=slice
      settings: infoedit="Extracts a given range of bits from each input sample and presents it at the output.  The output type is ordinarily unsigned with binary point at zero, but can be Boolean when the slice is one bit wide.<P><P>Hardware notes: In hardware this block costs nothing."  block_version=9.1.01
  Slice1 : xbsIndex_r4/Slice  nbits=1  boolean_output=off  mode=Upper Bit Location + Width  bit1=0  base1=MSB of Input  bit0=0  base0=LSB of Input  dbl_ovrd=off  block_type=slice
      settings: infoedit="Extracts a given range of bits from each input sample and presents it at the output.  The output type is ordinarily unsigned with binary point at zero, but can be Boolean when the slice is one bit wide.<P><P>Hardware notes: In hardware this block costs nothing."  block_version=9.1.01
  butterfly_direct : Subsystem  AncestorBlock=casper_library_ffts/butterfly_direct  mask(butterfly_direct){biplex=on, FFTSize=8, Coeffs=getfield( getfield( get_param( gcb,'UserData' ), 'parameters'),'Coeffs'), StepPeriod=2, coeff_bit_width=12, input_bit_width=12, downshift=off, add_latency=2, mult_latency=3, bram_latency=2, conv_latency=2, quantization=Round  (unbiased: +/- Inf), overflow=Saturate, arch=Virtex2Pro, opt_target=multipliers, coeffs_bram=on, use_hdl=on, use_embedded=off, hardcode_shifts=off, dsp48_adders=off}
      mask prompts: biplex "Used in biplex FFT"; FFTSize "Size of FFT: (2^? pts)"; Coeffs "Coefficients: (0 to 2^(FFTSize-1)-1)"; StepPeriod "Coefficient Step Period: (2^?)"; coeff_bit_width "Coefficient Bit Width"; input_bit_width "Input/Output Bit Width:"; add_latency "Add Latency"; mult_latency "Mult Latency"; bram_latency "BRAM Latency"; conv_latency "Convert latency"; quantization "Quantization Behavior"; overflow "Overflow Behavior"; arch "Architecture"; opt_target "Use less"; coeffs_bram "Store coefficients in BRAM"; use_hdl "Use behavioural HDL for multipliers"; use_embedded "Use embedded multipliers"; hardcode_shifts "Hardcode shift schedule"; dsp48_adders "Use DSP48s for adders"
      mask help: FFT internal block.
      mask init: same as fft_biplex_test/fft_biplex/biplex_core/fft_stage_1/butterfly_direct
      settings: AttributesFormatString=|
      | twiddle_general_3mult
      | coeffs in BRAM
      mask StyleString: checkbox,edit,edit,edit,edit,edit,checkbox,edit,edit,edit,edit,popup(Truncate|Round  (unbiased: +/- Inf)|Round  (unbiased: Even Values)),popup(Wrap|Saturate|Error),popup(Virtex2Pro|Virtex5),popup(logic|multipliers),checkbox,checkbox,checkbox,checkbox,checkbox
      mask CallbackString:
      | ||Coeffs = get_param(gcb, 'Coeffs');
      | if (length(eval(Coeffs)) == 1),
      |     set_param_state(gcb, 'StepPeriod', 'off');
      |     set_param_state(gcb, 'coeffs_bram', 'off');
      |     set_param_state(gcb, 'coeff_bit_width', 'off');
      | else
      |     set_param_state(gcb, 'StepPeriod', 'on');
      |     set_param_state(gcb, 'coeffs_bram', 'on');
      |     set_param_state(gcb, 'coeff_bit_width', 'on');
      | end|||||||||||fft_callback_arch(gcb);|||% make mutually exclusive with use_embedded.
      | 
      | use_hdl = get_param(gcb, 'use_hdl');
      | if strcmp(use_hdl, 'on'),
      |     set_param_state(gcb, 'use_embedded', 'off');
      | else
      |     set_param_state(gcb, 'use_embedded', 'on');
      | end|% make mutually exclusive with use_hdl.
      | 
      | use_hdl = get_param(gcb, 'use_embedded');
      | if strcmp(use_hdl, 'on'),
      |     set_param_state(gcb, 'use_hdl', 'off');
      | else
      |     set_param_state(gcb, 'use_hdl', 'on');
      | end|hardcode_shifts = get_param(gcb, 'hardcode_shifts');
      | set_param_state(gcb, 'downshift', hardcode_shifts);|fft_callback_dsp48_adders(gcb);
      mask TabNameString: Basic,Basic,Basic,Basic,Basic,Basic,Basic,Latency,Latency,Latency,Latency,Implementation,Implementation,Implementation,Implementation,Implementation,Implementation,Implementation,Implementation,Implementation
  delay_b : Subsystem  AncestorBlock=casper_library_delays/delay_bram  mask(delay_bram){DelayLen=2^(FFTSize-FFTStage), bram_latency=bram_latency, use_dsp48=off}
      mask prompts: DelayLen "Delay By:"; bram_latency "BRAM Latency"; use_dsp48 "Use DSP48"
      mask help: A delay block that uses BRAM for its storage.
      mask init: same as fft_biplex_test/fft_biplex/biplex_core/fft_stage_1/delay_b
      mask Help: eval('xlWeb(''http://casper.berkeley.edu/wiki/Delay_bram'')')
  delay_f : Subsystem  AncestorBlock=casper_library_delays/delay_bram  mask(delay_bram){DelayLen=2^(FFTSize-FFTStage), bram_latency=bram_latency, use_dsp48=off}
      mask prompts: DelayLen "Delay By:"; bram_latency "BRAM Latency"; use_dsp48 "Use DSP48"
      mask help: A delay block that uses BRAM for its storage.
      mask init: same as fft_biplex_test/fft_biplex/biplex_core/fft_stage_1/delay_b
      mask Help: eval('xlWeb(''http://casper.berkeley.edu/wiki/Delay_bram'')')
  sync_delay : casper_library_delays/sync_delay  SystemSampleTime=-1  DelayLen=2^(FFTSize - FFTStage)
  out1 : Outport  OutDataType=sfix(16)  OutScaling=2^0
  out2 : Outport  Port=2  OutDataType=sfix(16)  OutScaling=2^0
  of : Outport  Port=3  OutDataType=sfix(16)  OutScaling=2^0
  sync_out : Outport  Port=4  OutDataType=sfix(16)  OutScaling=2^0
  wires:
  shift/1 -> Slice/1
  of_in/1 -> Logical1/2
  Logical1/1 -> of/1
  Delay/1 -> sync_delay/1
  sync/1 -> Counter/1, Delay/1
  Counter/1 -> Slice1/1
  Mux/1 -> butterfly_direct/2(b)
  Mux1/1 -> delay_b/1(In1)
  delay_f/1(Out1) -> Mux1/3, Mux/2
  in1/1 -> Mux/3, Mux1/2
  Slice1/1 -> Mux/1, Mux1/1
  in2/1 -> delay_f/1(In1)
  delay_b/1(Out1) -> butterfly_direct/1(a)
  sync_delay/1 -> butterfly_direct/3(sync)
  Slice/1 -> butterfly_direct/4(shift)
  butterfly_direct/1(a+bw) -> out1/1
  butterfly_direct/2(a-bw) -> out2/1
  butterfly_direct/3(of) -> Logical1/1
  butterfly_direct/4(sync_out) -> sync_out/1
